simulink model "BESS_GFM_PV_GFL_10kV_Stage1"  (R2026a)
settings: Solver=ode23t  StopTime=0.8  MaxStep=1e-5
InitFcn:
  | run(fullfile(fileparts(get_param(bdroot,'FileName')),'..','scripts','init_bess_pv_stage1.m'));
undefined symbols (not defined in the file): ee_sli_rtmsupport, G, gcbh, S1
libraries: ee_lib x19, nesl_utility x15, fl_lib x14, eeGeneralControl x4, simulink x3, eeTransforms x2, sl_discontinuities x1, sl_signal_attributes x1
(part 1 of 2)
settings Model: Creator=fakebob2004  LastModifiedBy=fakebob2004
settings SimscapeCC: SimscapeLogType=none

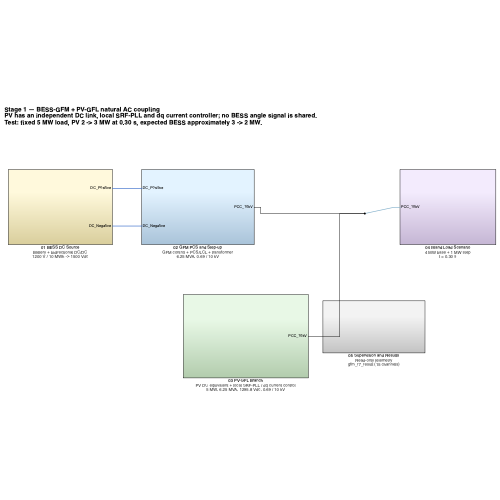
[thumbnail: Simulink's stored preview of the top-level diagram]
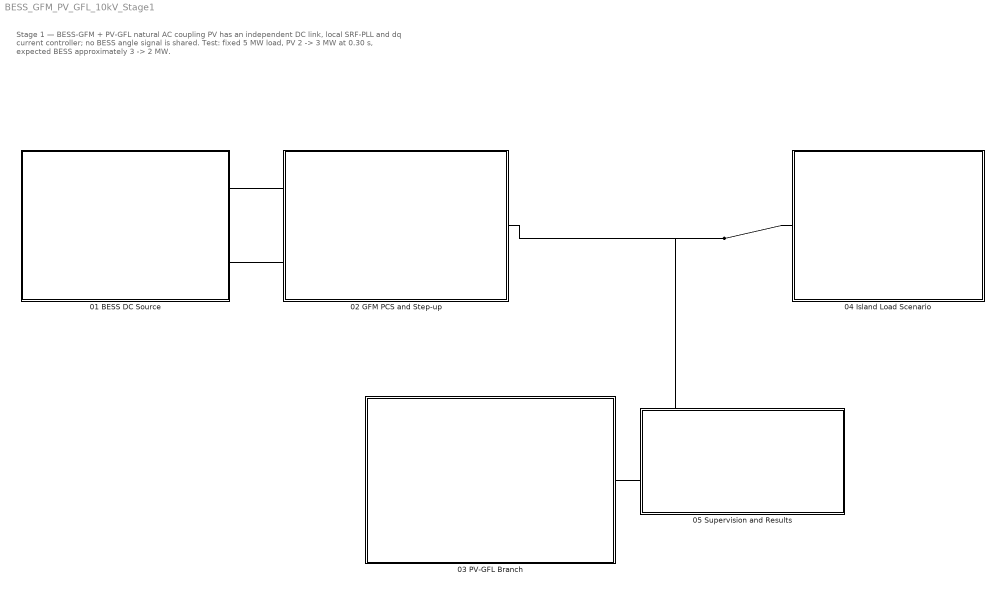
== system BESS_GFM_PV_GFL_10kV_Stage1 ==
  note: Stage 1 — BESS-GFM + PV-GFL natural AC coupling
      | PV has an independent DC link, local SRF-PLL and dq current controller; no BESS angle signal is shared.
      | Test: fixed 5 MW load, PV 2 -> 3 MW at 0.30 s, expected BESS approximately 3 -> 2 MW.
  01 BESS DC Source : Subsystem
      settings: AttributesFormatString=Battery + bidirectional DC/DC\n1200 V / 10 MWh -> 1500 Vdc
  02 GFM PCS and Step-up : Subsystem
      settings: AttributesFormatString=GFM control + PCS/LCL + transformer\n6.25 MVA, 0.69 / 10 kV
  03 PV-GFL Branch : Subsystem
      settings: AttributesFormatString=|
      | PV DC equivalent + local SRF-PLL / dq current control
      | 5 MW, 6.25 MVA, 1295.8 Vdc, 0.69 / 10 kV
  04 Island Load Scenario : Subsystem
      settings: AttributesFormatString=4 MW base + 1 MW step\nt = 0.30 s
  05 Supervision and Results : Subsystem
      settings: AttributesFormatString=Read-only telemetry\ngfm_r7_result (15 channels)
  connections:
  01 BESS DC Source/RConn1 -- 02 GFM PCS and Step-up/LConn1
  01 BESS DC Source/RConn2 -- 02 GFM PCS and Step-up/LConn2
  04 Island Load Scenario/LConn1 -- 02 GFM PCS and Step-up/RConn1 -- 03 PV-GFL Branch/RConn1

== system BESS_GFM_PV_GFL_10kV_Stage1/01 BESS DC Source ==
  01 Battery and DC Link : Subsystem
      settings: AttributesFormatString=1200 V / 10 MWh\n1500 V DC link
  02 Bidirectional DC-DC Control : Subsystem
      settings: AttributesFormatString=Vdc PI: 10 Hz\nIbat PI: 300 Hz
  DC_Positive : PMIOPort  Side=Right  ConnectionType=Connection: foundation.electrical.electrical
  DC_Negative : PMIOPort  Port=2  Side=Right  ConnectionType=Connection: foundation.electrical.electrical
  connections:
  02 Bidirectional DC-DC Control/RConn1 -- 01 Battery and DC Link/LConn2
  01 Battery and DC Link/RConn2 -- DC_Negative/RConn1
  DC_Positive/RConn1 -- 01 Battery and DC Link/LConn1

== system BESS_GFM_PV_GFL_10kV_Stage1/02 GFM PCS and Step-up ==
  03 GFM Control and Limits : Subsystem
      settings: AttributesFormatString=P-f / Q-V / Virtual Z\nAC limit: 1.20 pu
  04 PCS Filter and Transformer : Subsystem
      settings: AttributesFormatString=6.25 MVA PCS + LCL\n0.69 / 10 kV transformer
  DC_Positive : PMIOPort  Side=Left  ConnectionType=Connection: foundation.electrical.electrical
  DC_Negative : PMIOPort  Port=2  Side=Left  ConnectionType=Connection: foundation.electrical.electrical
  PCC_10kV : PMIOPort  Port=3  Side=Right  ConnectionType=Connection: foundation.electrical.three_phase
  connections:
  04 PCS Filter and Transformer/RConn3 -- DC_Negative/RConn1
  04 PCS Filter and Transformer/RConn2 -- PCC_10kV/RConn1
  04 PCS Filter and Transformer/RConn1 -- DC_Positive/RConn1
  03 GFM Control and Limits/RConn1 -- 04 PCS Filter and Transformer/LConn1

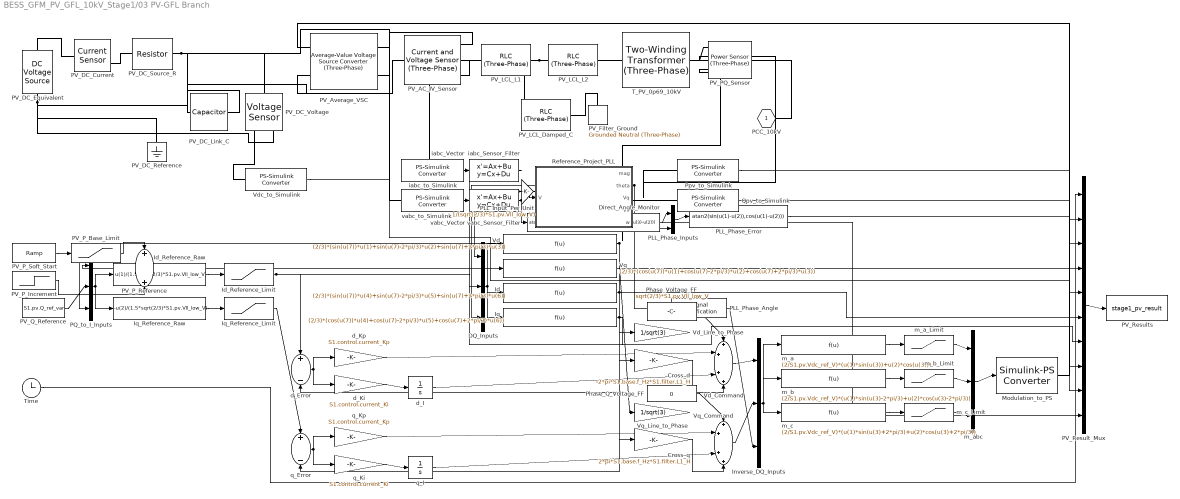
== system BESS_GFM_PV_GFL_10kV_Stage1/03 PV-GFL Branch ==
  Cross_d : Gain  Gain=-2*pi*S1.base.f_Hz*S1.filter.L1_H
  Cross_q : Gain  Gain=2*pi*S1.base.f_Hz*S1.filter.L1_H
  DQ_Inputs : Mux  Inputs=3
  Direct_Angle_Monitor : Fcn  Expr=atan2((2/3)*(u(1)-0.5*u(2)-0.5*u(3)),(sqrt(3)/3)*(u(3)-u(2)))
  Id : Fcn  Expr=(2/3)*(sin(u(7))*u(4)+sin(u(7)-2*pi/3)*u(5)+sin(u(7)+2*pi/3)*u(6))
  Id_Reference_Limit : Saturate  UpperLimit=S1.control.Ilimit_A  LowerLimit=-S1.control.Ilimit_A
  Id_Reference_Raw : Fcn  Expr=u(1)/(1.5*sqrt(2/3)*S1.pv.Vll_low_V)
  Inverse_DQ_Inputs : Mux  Inputs=3
  Iq : Fcn  Expr=(2/3)*(cos(u(7))*u(4)+cos(u(7)-2*pi/3)*u(5)+cos(u(7)+2*pi/3)*u(6))
  Iq_Reference_Limit : Saturate  UpperLimit=S1.control.Ilimit_A  LowerLimit=-S1.control.Ilimit_A
  Iq_Reference_Raw : Fcn  Expr=-u(2)/(1.5*sqrt(2/3)*S1.pv.Vll_low_V)
  Modulation_to_PS : nesl_utility/Simulink-PS Converter  PhysicalDomain=network_engine_domain  SubClassName=ps_input  LeftPortType=input  RightPortType=output  PseudoPeriodic=off  Frequencies=[]  NoiseDistribution=none  NoiseParameters=[]  Unit=1  AffineConversion=off  FilteringAndDerivatives=zero  SimscapeFilterOrder=1  InputFilterTimeConstant=0.001  UdotUserProvided=0
  PLL_Input_Per_Unit : Gain  Gain=1/(sqrt(2/3)*S1.pv.Vll_low_V)
  PLL_Phase_Angle : SignalSpecification
  PLL_Phase_Error : Fcn  Expr=atan2(sin(u(1)-u(2)),cos(u(1)-u(2)))
  PLL_Phase_Inputs : Mux  Inputs=2
  PQ_to_I_Inputs : Mux  Inputs=3
  PV_AC_IV_Sensor : ee_lib/Sensors & Transducers/Current and Voltage Sensor (Three-Phase)  port_option=ee.enum.threePhasePort.composite  vMeasurementType=ee.enum.vmeasurement.ll  outputUnit=ee.enum.unit.si  SRated=100e6 A*V  VRated=24e3 V  I_specify=off  I_priority=None  I=[0, 0, 0] A  I_nominal_specify=off  I_nominal_value=1  I_nominal_unit=A  V_specify=off  V_priority=None  V=[0, 0, 0] V  V_nominal_specify=off  V_nominal_value=1  V_nominal_unit=V
  PV_Average_VSC : ee_lib/Semiconductors & Converters/Converters/Average-Value Voltage Source Converter (Three-Phase)  port_option=ee.enum.threePhasePort.composite  enable_block_pulses_input=false  krec=0.001 Ohm  frequency_option=ee.enum.converters.frequency.variable  input_option=ee.enum.converters.inputOption.ModWave  FRated=S1.base.f_Hz Hz  losses_parameterization=ee.enum.converters.losses.fixed  Pfixed=1 W  ks=0.01  kc1=1.7 V  kc2=0.01 Ohm  Ploss_vect=[100, 800, 1870, 3250, 4900] W  Irms_vect=[10, 100, 200, 300, 400] A  Vdc_nom=300 V  thermal_mass=30000 J/K  temperature_specify=off  temperature_priority=High  temperature=298.15 K  temperature_nominal_specify=off  temperature_nominal_value=1  temperature_nominal_unit=K
  PV_DC_Current : fl_lib/Electrical/Electrical Sensors/Current Sensor
  PV_DC_Equivalent : fl_lib/Electrical/Electrical Sources/DC Voltage Source  v0=S1.pv.Vdc_ref_V V
  PV_DC_Link_C : fl_lib/Electrical/Electrical Elements/Capacitor  c=S1.pv.Cdc_F F  r=1e-6 Ohm  g=0 1/Ohm  i_specify=off  i_priority=None  i=0 A  i_nominal_specify=off  i_nominal_value=1  i_nominal_unit=A  v_specify=off  v_priority=None  v=0 V  v_nominal_specify=off  v_nominal_value=1  v_nominal_unit=V  vc_specify=on  vc_priority=High  vc=S1.pv.Vdc_ref_V V  vc_nominal_specify=off  vc_nominal_value=1  vc_nominal_unit=V
  PV_DC_Reference : fl_lib/Electrical/Electrical Elements/Electrical Reference
  PV_DC_Source_R : fl_lib/Electrical/Electrical Elements/Resistor  R=S1.pv.dc_source_R_ohm Ohm  i_specify=off  i_priority=None  i=0 A  i_nominal_specify=off  i_nominal_value=1  i_nominal_unit=A  v_specify=off  v_priority=None  v=0 V  v_nominal_specify=off  v_nominal_value=1  v_nominal_unit=V
  PV_DC_Voltage : fl_lib/Electrical/Electrical Sensors/Voltage Sensor
  PV_Filter_Ground : ee_lib/Connectors & References/Grounded Neutral (Three-Phase)  port_option=ee.enum.threePhasePort.composite
  PV_LCL_Damped_C : ee_lib/Passive/RLC Assemblies/RLC (Three-Phase)  port_option=ee.enum.threePhasePort.composite  component_structure=ee.enum.rlc.structure.SeriesRC  R=S1.filter.Rd_ohm Ohm  L=1e-3 H  C=S1.filter.C_F F  R_parasitic=0 Ohm  G_parasitic=0 1/Ohm  IL_specify=off  IL_priority=High  IL=[0, 0, 0] A  IL_nominal_specify=off  IL_nominal_value=1  IL_nominal_unit=A  VC_specify=off  VC_priority=High  VC=[0, 0, 0] V  VC_nominal_specify=off  VC_nominal_value=1  VC_nominal_unit=V
  PV_LCL_L1 : ee_lib/Passive/RLC Assemblies/RLC (Three-Phase)  port_option=ee.enum.threePhasePort.composite  component_structure=ee.enum.rlc.structure.SeriesRL  R=S1.filter.R1_ohm Ohm  L=S1.filter.L1_H H  C=1e-6 F  R_parasitic=0 Ohm  G_parasitic=0 1/Ohm  IL_specify=off  IL_priority=High  IL=[0, 0, 0] A  IL_nominal_specify=off  IL_nominal_value=1  IL_nominal_unit=A  VC_specify=off  VC_priority=High  VC=[0, 0, 0] V  VC_nominal_specify=off  VC_nominal_value=1  VC_nominal_unit=V
  PV_LCL_L2 : ee_lib/Passive/RLC Assemblies/RLC (Three-Phase)  port_option=ee.enum.threePhasePort.composite  component_structure=ee.enum.rlc.structure.SeriesRL  R=S1.filter.R2_ohm Ohm  L=S1.filter.L2_H H  C=1e-6 F  R_parasitic=0 Ohm  G_parasitic=0 1/Ohm  IL_specify=off  IL_priority=High  IL=[0, 0, 0] A  IL_nominal_specify=off  IL_nominal_value=1  IL_nominal_unit=A  VC_specify=off  VC_priority=High  VC=[0, 0, 0] V  VC_nominal_specify=off  VC_nominal_value=1  VC_nominal_unit=V
  PV_PQ_Sensor : ee_lib/Sensors & Transducers/Power Sensor (Three-Phase)  port_option=ee.enum.threePhasePort.composite  load_type=ee.enum.passive.type_balanced.balanced  f0=60 Hz
  PV_P_Base_Limit : Saturate  UpperLimit=S1.pv.P_initial_W  LowerLimit=0
  PV_P_Increment : Step  Time=S1.pv.P_step_time_s  FinalValue=S1.pv.P_final_W-S1.pv.P_initial_W  SampleTime=0
  PV_P_Reference : Sum
  PV_P_Soft_Start : simulink/Sources/Ramp  slope=S1.pv.P_ramp_W_per_s  start=0  InitialOutput=0
  PV_Q_Reference : Constant  Value=S1.pv.Q_ref_var
  PV_Result_Mux : Mux  Inputs=10
  PV_Results : ToWorkspace  VariableName=stage1_pv_result  SampleTime=-1
  Phase_Q_Voltage_FF : Constant  Value=0
  Phase_Voltage_FF : Constant  Value=sqrt(2/3)*S1.pv.Vll_low_V
  Ppv_to_Simulink : nesl_utility/PS-Simulink Converter  PhysicalDomain=network_engine_domain  SubClassName=ps_output  LeftPortType=input  RightPortType=output  PseudoPeriodic=off  Frequencies=[]  VectorFormat=inherit  Unit=W  AffineConversion=off
  Qpv_to_Simulink : nesl_utility/PS-Simulink Converter  PhysicalDomain=network_engine_domain  SubClassName=ps_output  LeftPortType=input  RightPortType=output  PseudoPeriodic=off  Frequencies=[]  VectorFormat=inherit  Unit=W  AffineConversion=off
  Reference_Project_PLL : Subsystem
      settings: PortSchema="{\"entries\":[{\"content\":{\"sides\":[{\"content\":{\"connectorIds\":[\"Out1\",\"Out2\",\"Out3\",\"Out4\",\"Out5\"]},\"type\":\"ConnectorPlacement.EquallySpacedRectSide\",\"uuid\":\"76485780-20fe-4fcf-8224-69648da6ed2a\"},{\"content\":{\"connectorIds\":[\"In1\"],\"side\":\"RIGHT\"},\"type\":\"ConnectorPlacement.EquallySpacedRectSide\",\"uuid\":\"f19a6390-e634-42c7-8d46-4cd80cbab182\"},{\"content\":{\"side\":\"TOP\"},\"type\":\"ConnectorPlacement.EquallySpacedRectSide\",\"uuid\":\"87682f72-1844-428e-be70-ad7ca3191ee3\"}]},\"type\":\"ConnectorPlacement.EquallySpacedConnector\",\"uuid\":\"f2136b07-48ec-402b-adb3-18c0bac2157c\"}],\"packageUris\":[\"http://schema.mathworks.com/mf0/Connector/R2020b\"],\"version\":\"1.0\"}"
  T_PV_0p69_10kV : ee_lib/Passive/Transformers/Two-Winding Transformer (Three-Phase)  SRated=S1.transformer.S_VA A*V  FRated=S1.base.f_Hz Hz  Winding1Connection=ee.enum.windingconnection.delta1  VRated1=S1.pv.Vll_low_V V  Winding2Connection=ee.enum.windingconnection.Yg  VRated2=S1.pv.Vll_high_V V  CoreType=ee.enum.coretype.threelimb  pu_Rw1=S1.transformer.R_pu/2  pu_Rw2=S1.transformer.R_pu/2  leakage_reactance_option=ee.enum.transformer_leakage.include  pu_Xl1=S1.transformer.X_pu/2  pu_Xl2=S1.transformer.X_pu/2  magnetizing_resistance_option=ee.enum.transformer_magnetizingResistance.exclude  pu_Rm=500  magnetizing_reactance_option=ee.enum.transformer_magnetizingReactance.exclude  saturation_option=ee.enum.transformer_saturation.exclude  pu_Xm=500  current_data=[0, .002, 1, 2]  magnetic_flux_data=[0, 1.2, 1.5, 1.51]  pu_X0=0.5  i1_specify=off  i1_priority=None  i1=[0, 0, 0] A  i1_nominal_specify=off  i1_nominal_value=1  i1_nominal_unit=A  i2_specify=off  i2_priority=None  i2=[0, 0, 0] A  i2_nominal_specify=off  i2_nominal_value=1  i2_nominal_unit=A  phi_specify=off  phi_priority=None  phi=[0, 0, 0]  phi_nominal_specify=off  phi_nominal_value=1  phi_nominal_unit=1
  Time : Clock
  Vd : Fcn  Expr=(2/3)*(sin(u(7))*u(1)+sin(u(7)-2*pi/3)*u(2)+sin(u(7)+2*pi/3)*u(3))
  Vd_Command : Sum  Inputs=++++
  Vd_Line_to_Phase : Gain  Gain=1/sqrt(3)
  Vdc_to_Simulink : nesl_utility/PS-Simulink Converter  PhysicalDomain=network_engine_domain  SubClassName=ps_output  LeftPortType=input  RightPortType=output  PseudoPeriodic=off  Frequencies=[]  VectorFormat=inherit  Unit=V  AffineConversion=off
  Vq : Fcn  Expr=(2/3)*(cos(u(7))*u(1)+cos(u(7)-2*pi/3)*u(2)+cos(u(7)+2*pi/3)*u(3))
  Vq_Command : Sum  Inputs=++++
  Vq_Line_to_Phase : Gain  Gain=1/sqrt(3)
  d_Error : Sum  Inputs=+-
  d_I : Integrator
  d_Ki : Gain  Gain=S1.control.current_Ki
  d_Kp : Gain  Gain=S1.control.current_Kp
  iabc_Sensor_Filter : StateSpace  A=-eye(3)/S1.control.sensor_filter_s  B=eye(3)/S1.control.sensor_filter_s  C=eye(3)  D=zeros(3)  InitialCondition=zeros(3,1)
  iabc_Vector : Reshape
  iabc_to_Simulink : nesl_utility/PS-Simulink Converter  PhysicalDomain=network_engine_domain  SubClassName=ps_output  LeftPortType=input  RightPortType=output  PseudoPeriodic=off  Frequencies=[]  VectorFormat=inherit  Unit=A  AffineConversion=off
  m_a : Fcn  Expr=(2/S1.pv.Vdc_ref_V)*(u(1)*sin(u(3))+u(2)*cos(u(3)))
  m_a_Limit : Saturate  UpperLimit=S1.pv.modulation_max  LowerLimit=-S1.pv.modulation_max
  m_abc : Mux  Inputs=3
  m_b : Fcn  Expr=(2/S1.pv.Vdc_ref_V)*(u(1)*sin(u(3)-2*pi/3)+u(2)*cos(u(3)-2*pi/3))
  m_b_Limit : Saturate  UpperLimit=S1.pv.modulation_max  LowerLimit=-S1.pv.modulation_max
  m_c : Fcn  Expr=(2/S1.pv.Vdc_ref_V)*(u(1)*sin(u(3)+2*pi/3)+u(2)*cos(u(3)+2*pi/3))
  m_c_Limit : Saturate  UpperLimit=S1.pv.modulation_max  LowerLimit=-S1.pv.modulation_max
  q_Error : Sum  Inputs=+-
  q_I : Integrator
  q_Ki : Gain  Gain=S1.control.current_Ki
  q_Kp : Gain  Gain=S1.control.current_Kp
  vabc_Sensor_Filter : StateSpace  A=-eye(3)/S1.control.sensor_filter_s  B=eye(3)/S1.control.sensor_filter_s  C=eye(3)  D=zeros(3)  InitialCondition=sqrt(2/3)*S1.pv.Vll_low_V*[sin(pi/6);sin(pi/6-2*pi/3);sin(pi/6+2*pi/3)]
  vabc_Vector : Reshape
  vabc_to_Simulink : nesl_utility/PS-Simulink Converter  PhysicalDomain=network_engine_domain  SubClassName=ps_output  LeftPortType=input  RightPortType=output  PseudoPeriodic=off  Frequencies=[]  VectorFormat=inherit  Unit=V  AffineConversion=off
  PCC_10kV : PMIOPort  Side=Right  ConnectionType=Connection: foundation.electrical.three_phase
  wires:
  iabc_to_Simulink/1 -> iabc_Vector/1
  vabc_to_Simulink/1 -> vabc_Vector/1
  iabc_Vector/1 -> iabc_Sensor_Filter/1
  vabc_Vector/1 -> vabc_Sensor_Filter/1
  vabc_Sensor_Filter/1 -> PLL_Input_Per_Unit/1, Direct_Angle_Monitor/1, DQ_Inputs/1
  PLL_Input_Per_Unit/1 -> Reference_Project_PLL/1(V)
  Direct_Angle_Monitor/1 -> PLL_Phase_Inputs/1
  Reference_Project_PLL/2(theta) -> PLL_Phase_Inputs/2, DQ_Inputs/3, PLL_Phase_Angle/1
  PLL_Phase_Inputs/1 -> PLL_Phase_Error/1
  iabc_Sensor_Filter/1 -> DQ_Inputs/2
  DQ_Inputs/1 -> Vd/1, Vq/1, Id/1, Iq/1
  PV_P_Soft_Start/1 -> PV_P_Base_Limit/1
  PV_P_Base_Limit/1 -> PV_P_Reference/1
  PV_P_Increment/1 -> PV_P_Reference/2
  PV_P_Reference/1 -> PQ_to_I_Inputs/1, PV_Result_Mux/4
  PV_Q_Reference/1 -> PQ_to_I_Inputs/2
  Vd/1 -> PQ_to_I_Inputs/3, Vd_Line_to_Phase/1
  PQ_to_I_Inputs/1 -> Id_Reference_Raw/1, Iq_Reference_Raw/1
  Id_Reference_Raw/1 -> Id_Reference_Limit/1
  Iq_Reference_Raw/1 -> Iq_Reference_Limit/1
  d_Error/1 -> d_Kp/1, d_Ki/1
  d_Ki/1 -> d_I/1
  q_Error/1 -> q_Kp/1, q_Ki/1
  q_Ki/1 -> q_I/1
  Id_Reference_Limit/1 -> d_Error/1, PV_Result_Mux/8
  Id/1 -> d_Error/2, Cross_q/1, PV_Result_Mux/6
  Iq_Reference_Limit/1 -> q_Error/1
  Iq/1 -> q_Error/2, Cross_d/1, PV_Result_Mux/7
  Vq/1 -> Vq_Line_to_Phase/1
  Phase_Voltage_FF/1 -> Vd_Command/1
  d_Kp/1 -> Vd_Command/2
  d_I/1 -> Vd_Command/3
  Cross_d/1 -> Vd_Command/4
  Phase_Q_Voltage_FF/1 -> Vq_Command/1
  q_Kp/1 -> Vq_Command/2
  q_I/1 -> Vq_Command/3
  Cross_q/1 -> Vq_Command/4
  Vd_Command/1 -> Inverse_DQ_Inputs/1
  Vq_Command/1 -> Inverse_DQ_Inputs/2
  PLL_Phase_Angle/1 -> Inverse_DQ_Inputs/3
  Inverse_DQ_Inputs/1 -> m_a/1, m_b/1, m_c/1
  m_a/1 -> m_a_Limit/1
  m_b/1 -> m_b_Limit/1
  m_c/1 -> m_c_Limit/1
  m_a_Limit/1 -> m_abc/1
  m_b_Limit/1 -> m_abc/2
  m_c_Limit/1 -> m_abc/3
  m_abc/1 -> Modulation_to_PS/1
  Time/1 -> PV_Result_Mux/1
  Ppv_to_Simulink/1 -> PV_Result_Mux/2
  Qpv_to_Simulink/1 -> PV_Result_Mux/3
  PLL_Phase_Error/1 -> PV_Result_Mux/5
  Vdc_to_Simulink/1 -> PV_Result_Mux/9
  Reference_Project_PLL/5(w) -> PV_Result_Mux/10
  PV_Result_Mux/1 -> PV_Results/1
  connections:
  PV_DC_Equivalent/LConn1 -- PV_DC_Current/LConn1
  PV_DC_Current/RConn2 -- PV_DC_Source_R/LConn1
  PV_Average_VSC/RConn1 -- PV_DC_Source_R/RConn1 -- PV_DC_Link_C/LConn1 -- PV_DC_Voltage/LConn1
  PV_Average_VSC/RConn2 -- PV_DC_Equivalent/RConn1 -- PV_DC_Link_C/RConn1 -- PV_DC_Voltage/RConn2 -- PV_DC_Reference/LConn1
  PV_Average_VSC/LConn2 -- PV_AC_IV_Sensor/LConn1
  PV_AC_IV_Sensor/RConn3 -- PV_LCL_L1/LConn1
  PV_LCL_L2/LConn1 -- PV_LCL_L1/RConn1 -- PV_LCL_Damped_C/LConn1
  PV_LCL_Damped_C/RConn1 -- PV_Filter_Ground/LConn1
  PV_LCL_L2/RConn1 -- T_PV_0p69_10kV/LConn1
  T_PV_0p69_10kV/RConn1 -- PV_PQ_Sensor/LConn1
  PV_PQ_Sensor/RConn1 -- PCC_10kV/RConn1
  PV_AC_IV_Sensor/RConn2 -- iabc_to_Simulink/LConn1
  PV_AC_IV_Sensor/RConn1 -- vabc_to_Simulink/LConn1
  PV_PQ_Sensor/LConn2 -- Ppv_to_Simulink/LConn1
  PV_PQ_Sensor/LConn3 -- Qpv_to_Simulink/LConn1
  PV_DC_Voltage/RConn1 -- Vdc_to_Simulink/LConn1
  Modulation_to_PS/RConn1 -- PV_Average_VSC/LConn1

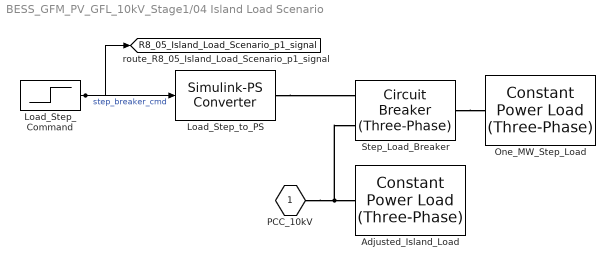
== system BESS_GFM_PV_GFL_10kV_Stage1/04 Island Load Scenario ==
  Adjusted_Island_Load : ee_lib/Passive/Constant Power Load (Three-Phase)  port_option=ee.enum.threePhasePort.composite  FRated=G.f0_Hz Hz  active_power=S1.load.P_W W  reactive_power=S1.load.Q_var V*A  Vline_rms_min=0.70*G.ac.Vll_high_V V  tau=0.01 s  Vline_rms_ini=G.ac.Vll_high_V V  Vang_ini=0 deg  gmin=1e-6 S
  Load_Step_Command : Step  Time=G.load.step_time_s  InitialValue=1  FinalValue=0  SampleTime=0
  Load_Step_to_PS : nesl_utility/Simulink-PS Converter  PhysicalDomain=network_engine_domain  SubClassName=ps_input  LeftPortType=input  RightPortType=output  PseudoPeriodic=off  Frequencies=[]  NoiseDistribution=none  NoiseParameters=[]  Unit=V  AffineConversion=off  FilteringAndDerivatives=zero  SimscapeFilterOrder=1  InputFilterTimeConstant=0.001  UdotUserProvided=0
  One_MW_Step_Load : ee_lib/Passive/Constant Power Load (Three-Phase)  port_option=ee.enum.threePhasePort.composite  FRated=G.f0_Hz Hz  active_power=0 W  reactive_power=0 V*A  Vline_rms_min=0.70*G.ac.Vll_high_V V  tau=0.01 s  Vline_rms_ini=G.ac.Vll_high_V V  Vang_ini=0 deg  gmin=1e-6 S
  Step_Load_Breaker : ee_lib/Switches & Breakers/Circuit Breaker (Three-Phase)  port_option=ee.enum.threePhasePort.composite  control_port_option=ee.enum.controlport.ps  R_closed=0.001 Ohm  G_open=1e-6 1/Ohm  threshold=0.5 V  breaker_behavior=ee.enum.switches.breakerBehavior.zeroCrossingEnable  i_th=1e-8 A
  PCC_10kV : PMIOPort  Side=Left  ConnectionType=Connection: foundation.electrical.three_phase
  tag scope: R8_05_Island_Load_Scenario_p1_signal=global
  wires:
  Load_Step_Command/1 -> Load_Step_to_PS/1, [R8_05_Island_Load_Scenario_p1_signal]  "step_breaker_cmd"
  connections:
  Step_Load_Breaker/RConn1 -- One_MW_Step_Load/LConn1
  PCC_10kV/RConn1 -- Adjusted_Island_Load/LConn1 -- Step_Load_Breaker/LConn2
  Load_Step_to_PS/RConn1 -- Step_Load_Breaker/LConn1

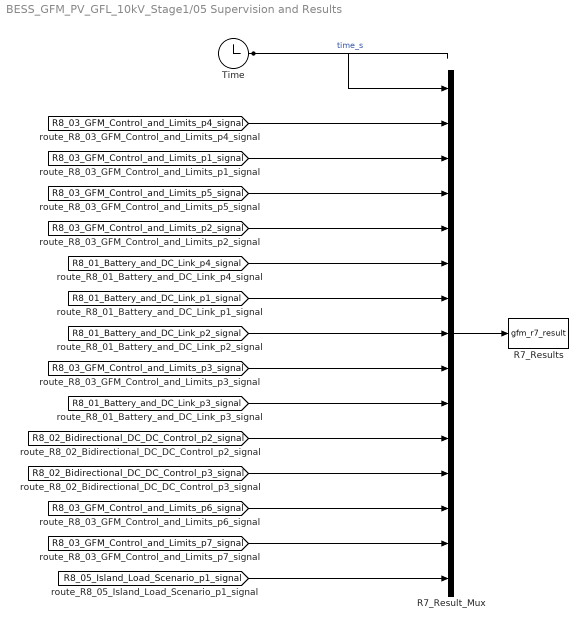
== system BESS_GFM_PV_GFL_10kV_Stage1/05 Supervision and Results ==
  R7_Result_Mux : Mux  Inputs=15
  R7_Results : ToWorkspace  VariableName=gfm_r7_result  SampleTime=-1
  Time : Clock
  wires:
  [R8_05_Island_Load_Scenario_p1_signal] -> R7_Result_Mux/15
  [R8_03_GFM_Control_and_Limits_p7_signal] -> R7_Result_Mux/14
  R7_Result_Mux/1 -> R7_Results/1
  [R8_03_GFM_Control_and_Limits_p6_signal] -> R7_Result_Mux/13
  [R8_02_Bidirectional_DC_DC_Control_p3_signal] -> R7_Result_Mux/12
  [R8_02_Bidirectional_DC_DC_Control_p2_signal] -> R7_Result_Mux/11
  [R8_01_Battery_and_DC_Link_p3_signal] -> R7_Result_Mux/10
  [R8_03_GFM_Control_and_Limits_p3_signal] -> R7_Result_Mux/9
  [R8_01_Battery_and_DC_Link_p2_signal] -> R7_Result_Mux/8
  [R8_01_Battery_and_DC_Link_p1_signal] -> R7_Result_Mux/7
  [R8_01_Battery_and_DC_Link_p4_signal] -> R7_Result_Mux/6
  [R8_03_GFM_Control_and_Limits_p2_signal] -> R7_Result_Mux/5
  Time/1 -> R7_Result_Mux/1  "time_s"
  [R8_03_GFM_Control_and_Limits_p5_signal] -> R7_Result_Mux/4
  [R8_03_GFM_Control_and_Limits_p1_signal] -> R7_Result_Mux/3
  [R8_03_GFM_Control_and_Limits_p4_signal] -> R7_Result_Mux/2

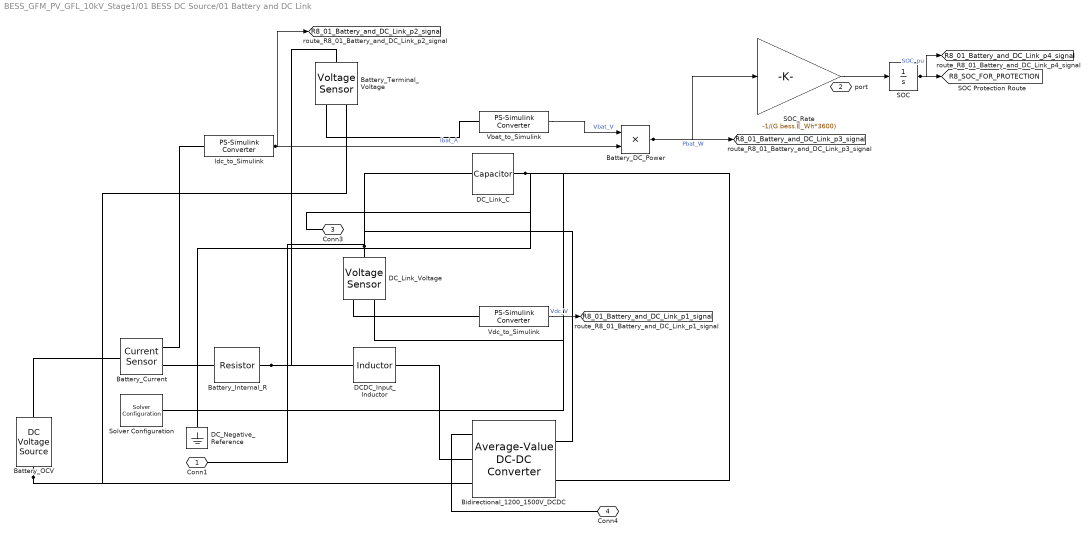
== system BESS_GFM_PV_GFL_10kV_Stage1/01 BESS DC Source/01 Battery and DC Link ==
  Battery_Current : fl_lib/Electrical/Electrical Sensors/Current Sensor
  Battery_DC_Power : Product
  Battery_Internal_R : fl_lib/Electrical/Electrical Elements/Resistor  R=G.dc.Rbattery_ohm Ohm  i_specify=off  i_priority=None  i=0 A  i_nominal_specify=off  i_nominal_value=1  i_nominal_unit=A  v_specify=off  v_priority=None  v=0 V  v_nominal_specify=off  v_nominal_value=1  v_nominal_unit=V
  Battery_OCV : fl_lib/Electrical/Electrical Sources/DC Voltage Source  v0=G.dc.Vbattery_V V
  Battery_Terminal_Voltage : fl_lib/Electrical/Electrical Sensors/Voltage Sensor
  Bidirectional_1200_1500V_DCDC : ee_lib/Semiconductors & Converters/Converters/Average-Value DC-DC Converter  implementation_option=ee.enum.converters.implementation.behavioral  converter_type=ee.enum.converters.dcdctype.buckboost  control_option=ee.enum.converters.controlinput.dutycycle  efficiency_option=ee.enum.converters.efficiency.constant  efficiency_fixed=G.dc.dcdc_efficiency_pct  i_vec=[0, 2, 5] A  efficiency_vec=[90, 95, 98]  Lf=1e-6 H  Rl=0 Ohm  Cf=1e-7 F  Rc=1e-6 Ohm  iL_specify=off  iL_priority=High  iL=0 A  iL_nominal_specify=off  iL_nominal_value=1  iL_nominal_unit=A  vc_specify=off  vc_priority=High  vc=0 V  vc_nominal_specify=off  vc_nominal_value=1  vc_nominal_unit=V
  DCDC_Input_Inductor : fl_lib/Electrical/Electrical Elements/Inductor  l=G.dcdc.L_H H  r=0 Ohm  g=1e-9 1/Ohm  i_specify=on  i_priority=None  i=G.dcdc.Iref_initial_A A  i_nominal_specify=off  i_nominal_value=1  i_nominal_unit=A  v_specify=off  v_priority=None  v=0 V  v_nominal_specify=off  v_nominal_value=1  v_nominal_unit=V  i_L_specify=off  i_L_priority=High  i_L=0 A  i_L_nominal_specify=off  i_L_nominal_value=1  i_L_nominal_unit=A
  DC_Link_C : fl_lib/Electrical/Electrical Elements/Capacitor  c=G.dc.Cdc_F F  r=1e-6 Ohm  g=0 1/Ohm  i_specify=off  i_priority=None  i=0 A  i_nominal_specify=off  i_nominal_value=1  i_nominal_unit=A  v_specify=off  v_priority=None  v=0 V  v_nominal_specify=off  v_nominal_value=1  v_nominal_unit=V  vc_specify=on  vc_priority=High  vc=G.dc.Vdc_ref_V V  vc_nominal_specify=off  vc_nominal_value=1  vc_nominal_unit=V
  DC_Link_Voltage : fl_lib/Electrical/Electrical Sensors/Voltage Sensor
  DC_Negative_Reference : fl_lib/Electrical/Electrical Elements/Electrical Reference
  Idc_to_Simulink : nesl_utility/PS-Simulink Converter  PhysicalDomain=network_engine_domain  SubClassName=ps_output  LeftPortType=input  RightPortType=output  PseudoPeriodic=off  Frequencies=[]  VectorFormat=inherit  Unit=A  AffineConversion=off
  SOC : Integrator  InitialCondition=G.bess.SOC0  LimitOutput=on  UpperSaturationLimit=G.bess.SOC_max  LowerSaturationLimit=G.bess.SOC_min
  SOC_Rate : Gain  Gain=-1/(G.bess.E_Wh*3600)
  Solver Configuration : nesl_utility/Solver Configuration  PhysicalDomain=network_engine_domain  SubClassName=solver  LeftPortType=input  RightPortType=generic  Tones=[]  Harmonics=[]  SimulateNoise=off  Profile=off  UseLocalSampling=off  EnableSwitchedLinearOptims=on  FrequencyDomain=off  UseCCode=off  RelTol=0.001  AbsTol=0.001  MinStep=1e-09  ToWorkspace=off  RevertToSquareIcSolve=off  NumHomotopyIterations=100  PhasorMode=off  PhasorModeNumHarmonics=1  ConsistencySolver=NEWTON_XTOL_AFTER_FTOL  CanonicalOrdering=CANONICAL  OptimizeIntermediates=OPTIMIZED  IndexReductionMethod=DerivativeReplacement  DoDC=off  ResidualTolerance=1e-09  ConsistencyTolSource=GLOBAL  ConsistencyAbsTol=0.001  ConsistencyRelTol=0.001  ConsistencyTolFactor=0.001  UseLocalSolver=off  LocalSolverChoice=NE_BACKWARD_EULER_ADVANCER  ResolveIndetEquations=on  FunctionEvalNumThread=1  LocalSolverSampleTime=0.001  DoFixedCost=off  MaxNonlinIter=3  MaxModeIter=2  ComputeImpulses=off  ImpulseIterations=2  LinearAlgebra=auto  LinearAlgebraNumThread=0  EquationFormulation=NE_TIME_EF  DelaysMemoryBudget=1024  AutomaticFiltering=on  FilteringTimeConstant=0.001  PartitionStorageMethod=AS_NEEDED  PartitionMemoryBudget=1024  PartitionMethod=ROBUST  MultibodyUseLocalSolver=off  MultibodyLocalSolverChoice=ODE1  MultibodyLocalSolverSampleTime=0.001
  Vbat_to_Simulink : nesl_utility/PS-Simulink Converter  PhysicalDomain=network_engine_domain  SubClassName=ps_output  LeftPortType=input  RightPortType=output  PseudoPeriodic=off  Frequencies=[]  VectorFormat=inherit  Unit=V  AffineConversion=off
  Vdc_to_Simulink : nesl_utility/PS-Simulink Converter  PhysicalDomain=network_engine_domain  SubClassName=ps_output  LeftPortType=input  RightPortType=output  PseudoPeriodic=off  Frequencies=[]  VectorFormat=inherit  Unit=V  AffineConversion=off
  Conn1 : PMIOPort  Side=Left
  port : PMIOPort  Port=2  Side=Right
  Conn3 : PMIOPort  Port=3  Side=Right
  Conn4 : PMIOPort  Port=4  Side=Left
  tag scope: R8_01_Battery_and_DC_Link_p1_signal=global, R8_01_Battery_and_DC_Link_p2_signal=global, R8_01_Battery_and_DC_Link_p3_signal=global, R8_01_Battery_and_DC_Link_p4_signal=global, R8_SOC_FOR_PROTECTION=global
  wires:
  SOC/1 -> [R8_01_Battery_and_DC_Link_p4_signal], [R8_SOC_FOR_PROTECTION]  "SOC_pu"
  Battery_DC_Power/1 -> SOC_Rate/1, [R8_01_Battery_and_DC_Link_p3_signal]  "Pbat_W"
  Vbat_to_Simulink/1 -> Battery_DC_Power/1  "Vbat_V"
  Vdc_to_Simulink/1 -> [R8_01_Battery_and_DC_Link_p1_signal]  "Vdc_V"
  SOC_Rate/1 -> SOC/1
  Idc_to_Simulink/1 -> [R8_01_Battery_and_DC_Link_p2_signal], Battery_DC_Power/2  "Ibat_A"
  connections:
  Conn4/RConn1 -- Bidirectional_1200_1500V_DCDC/LConn1
  DC_Link_Voltage/LConn1 -- Bidirectional_1200_1500V_DCDC/RConn1 -- DC_Link_C/LConn1 -- Conn1/RConn1
  Battery_Terminal_Voltage/RConn1 -- Vbat_to_Simulink/LConn1
  DC_Link_Voltage/RConn1 -- Vdc_to_Simulink/LConn1
  Battery_Internal_R/RConn1 -- DCDC_Input_Inductor/LConn1 -- Battery_Terminal_Voltage/LConn1
  Battery_Current/RConn2 -- Battery_Internal_R/LConn1
  DCDC_Input_Inductor/RConn1 -- Bidirectional_1200_1500V_DCDC/LConn2
  Battery_Current/RConn1 -- Idc_to_Simulink/LConn1
  Battery_OCV/LConn1 -- Battery_Current/LConn1
  DC_Negative_Reference/LConn1 -- DC_Link_C/RConn1 -- Bidirectional_1200_1500V_DCDC/RConn2 -- DC_Link_Voltage/RConn2 -- Conn3/RConn1 -- Solver Configuration/RConn1
  Battery_OCV/RConn1 -- Battery_Terminal_Voltage/RConn2 -- Bidirectional_1200_1500V_DCDC/LConn3

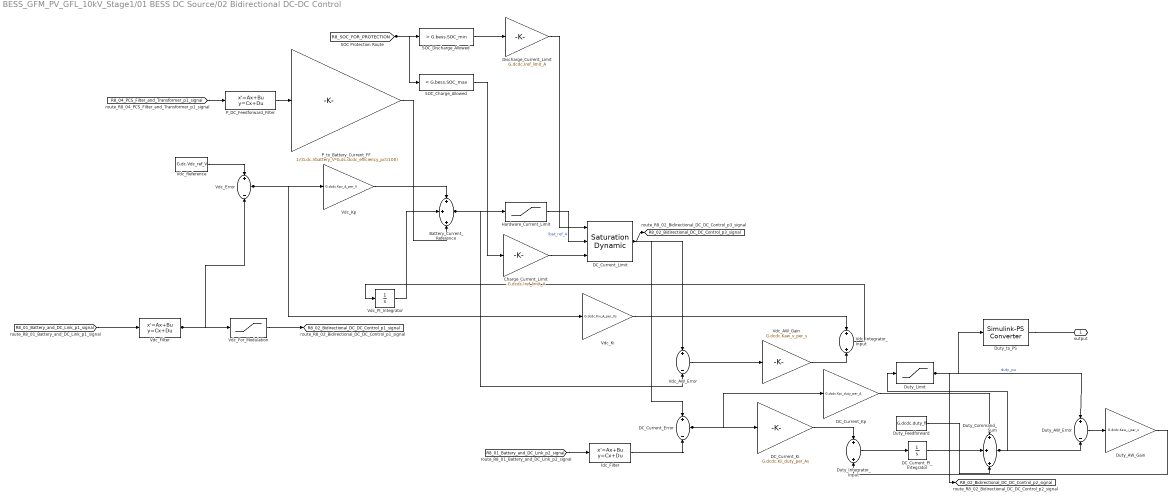
== system BESS_GFM_PV_GFL_10kV_Stage1/01 BESS DC Source/02 Bidirectional DC-DC Control ==
  Battery_Current_Reference : Sum  Inputs=+++
  Charge_Current_Limit : Gain  Gain=-G.dcdc.Iref_limit_A
  DC_Current_Error : Sum  Inputs=+-
  DC_Current_Ki : Gain  Gain=G.dcdc.Kii_duty_per_As
  DC_Current_Kp : Gain  Gain=G.dcdc.Kpi_duty_per_A
  DC_Current_Limit : sl_discontinuities/Saturation Dynamic  OutMin=[]  OutMax=[]  OutDataTypeStr=Inherit: Same as second input  OutDataType=fixdt(1, 16)  OutScaling=2^-10  DoSatur=off
      settings: LibrarySourceBlock=|
      | simulink/Discontinuities/Saturation
      | Dynamic
  DC_Current_PI_Integrator : Integrator
  Discharge_Current_Limit : Gain  Gain=G.dcdc.Iref_limit_A
  Duty_AW_Error : Sum  Inputs=+-
  Duty_AW_Gain : Gain  Gain=G.dcdc.Kaw_i_per_s
  Duty_Command_Sum : Sum  Inputs=+++
  Duty_Feedforward : Constant  Value=G.dcdc.duty_ff
  Duty_Integrator_Input : Sum
  Duty_Limit : Saturate  UpperLimit=G.dcdc.duty_max  LowerLimit=G.dcdc.duty_min
  Duty_to_PS : nesl_utility/Simulink-PS Converter  PhysicalDomain=network_engine_domain  SubClassName=ps_input  LeftPortType=input  RightPortType=output  PseudoPeriodic=off  Frequencies=[]  NoiseDistribution=none  NoiseParameters=[]  Unit=1  AffineConversion=off  FilteringAndDerivatives=zero  SimscapeFilterOrder=1  InputFilterTimeConstant=0.001  UdotUserProvided=0
  Hardware_Current_Limit : Saturate  UpperLimit=G.dcdc.Iref_limit_A  LowerLimit=-G.dcdc.Iref_limit_A
  Idc_Filter : StateSpace  A=-1/G.dcdc.current_sensor_s  B=1/G.dcdc.current_sensor_s  D=0  InitialCondition=G.dcdc.Iref_initial_A
  P_DC_Feedforward_Filter : StateSpace  A=-1/G.dcdc.power_ff_filter_s  B=1/G.dcdc.power_ff_filter_s  D=0  InitialCondition=G.load.base_P_W
  P_to_Battery_Current_FF : Gain  Gain=1/(G.dc.Vbattery_V*G.dc.dcdc_efficiency_pct/100)
  SOC_Charge_Allowed : simulink/Logic and Bit Operations/Compare To Constant  relop=<  const=G.bess.SOC_max  OutDataTypeStr=boolean
  SOC_Discharge_Allowed : simulink/Logic and Bit Operations/Compare To Constant  relop=>  const=G.bess.SOC_min  OutDataTypeStr=boolean
  Vdc_AW_Error : Sum  Inputs=+-
  Vdc_AW_Gain : Gain  Gain=G.dcdc.Kaw_v_per_s
  Vdc_Error : Sum  Inputs=+-
  Vdc_Filter : StateSpace  A=-1/G.control.Vdc_filter_s  B=1/G.control.Vdc_filter_s  D=0  InitialCondition=G.dc.Vdc_ref_V
  Vdc_For_Modulation : Saturate  UpperLimit=2000  LowerLimit=500
  Vdc_Integrator_Input : Sum
  Vdc_Ki : Gain  Gain=G.dcdc.Kiv_A_per_Vs
  Vdc_Kp : Gain  Gain=G.dcdc.Kpv_A_per_V
  Vdc_PI_Integrator : Integrator
  Vdc_Reference : Constant  Value=G.dc.Vdc_ref_V
  output : PMIOPort  Side=Right
  tag scope: R8_02_Bidirectional_DC_DC_Control_p1_signal=global, R8_02_Bidirectional_DC_DC_Control_p2_signal=global, R8_02_Bidirectional_DC_DC_Control_p3_signal=global
  wires:
  Duty_AW_Gain/1 -> Duty_Integrator_Input/2
  Duty_Limit/1 -> [R8_02_Bidirectional_DC_DC_Control_p2_signal], Duty_AW_Error/1, Duty_to_PS/1  "duty_pu"
  Duty_Integrator_Input/1 -> DC_Current_PI_Integrator/1
  DC_Current_Error/1 -> DC_Current_Ki/1, DC_Current_Kp/1
  Idc_Filter/1 -> DC_Current_Error/2
  Discharge_Current_Limit/1 -> DC_Current_Limit/1
  Vdc_Ki/1 -> Vdc_Integrator_Input/1
  SOC_Charge_Allowed/1 -> Charge_Current_Limit/1
  DC_Current_Limit/1 -> [R8_02_Bidirectional_DC_DC_Control_p3_signal], DC_Current_Error/1, Vdc_AW_Error/1
  [R8_01_Battery_and_DC_Link_p2_signal] -> Idc_Filter/1
  Vdc_AW_Error/1 -> Vdc_AW_Gain/1
  Charge_Current_Limit/1 -> DC_Current_Limit/3
  Hardware_Current_Limit/1 -> DC_Current_Limit/2  "Ibat_ref_A"
  Vdc_Integrator_Input/1 -> Vdc_PI_Integrator/1
  Battery_Current_Reference/1 -> Hardware_Current_Limit/1, Vdc_AW_Error/2
  DC_Current_PI_Integrator/1 -> Duty_Command_Sum/2
  SOC_Discharge_Allowed/1 -> Discharge_Current_Limit/1
  Vdc_PI_Integrator/1 -> Battery_Current_Reference/2
  [R8_04_PCS_Filter_and_Transformer_p1_signal] -> P_DC_Feedforward_Filter/1
  Duty_Feedforward/1 -> Duty_Command_Sum/3
  Vdc_For_Modulation/1 -> [R8_02_Bidirectional_DC_DC_Control_p1_signal]
  [R8_SOC_FOR_PROTECTION] -> SOC_Discharge_Allowed/1, SOC_Charge_Allowed/1
  Vdc_Error/1 -> Vdc_Kp/1, Vdc_Ki/1
  Duty_AW_Error/1 -> Duty_AW_Gain/1
  Vdc_AW_Gain/1 -> Vdc_Integrator_Input/2
  Vdc_Reference/1 -> Vdc_Error/1
  [R8_01_Battery_and_DC_Link_p1_signal] -> Vdc_Filter/1
  DC_Current_Ki/1 -> Duty_Integrator_Input/1
  P_DC_Feedforward_Filter/1 -> P_to_Battery_Current_FF/1
  Vdc_Kp/1 -> Battery_Current_Reference/1
  DC_Current_Kp/1 -> Duty_Command_Sum/1
  P_to_Battery_Current_FF/1 -> Battery_Current_Reference/3
  Duty_Command_Sum/1 -> Duty_AW_Error/2, Duty_Limit/1
  Vdc_Filter/1 -> Vdc_For_Modulation/1, Vdc_Error/2
  connections:
  Duty_to_PS/RConn1 -- output/RConn1

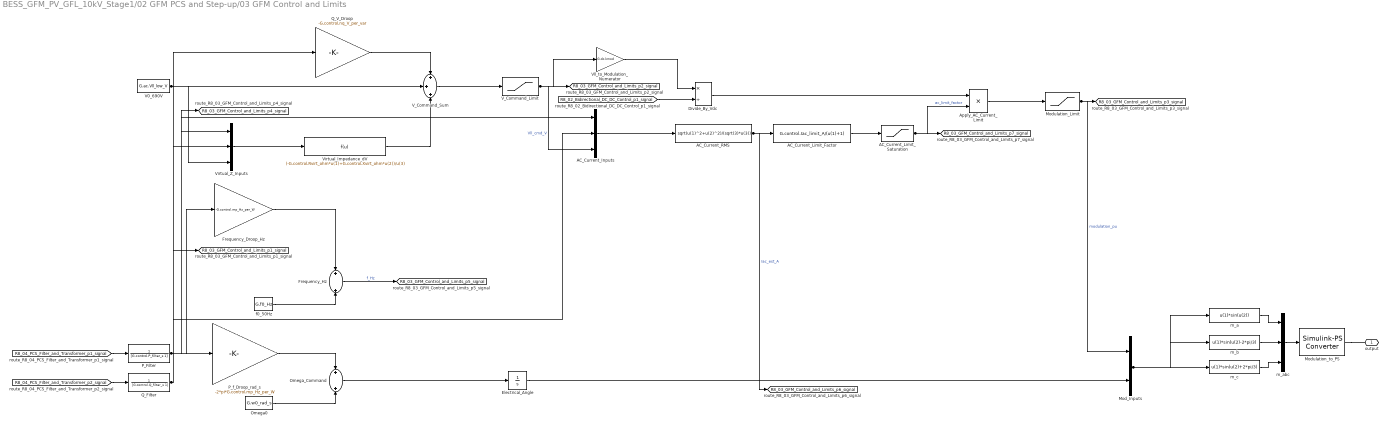
== system BESS_GFM_PV_GFL_10kV_Stage1/02 GFM PCS and Step-up/03 GFM Control and Limits ==
  AC_Current_Inputs : Mux  Inputs=3
  AC_Current_Limit_Factor : Fcn  Expr=G.control.Iac_limit_A/(u(1)+1)
  AC_Current_Limit_Saturation : Saturate  UpperLimit=1  LowerLimit=0
  AC_Current_RMS : Fcn  Expr=sqrt(u(1)^2+u(2)^2)/(sqrt(3)*u(3))
  Apply_AC_Current_Limit : Product
  Divide_By_Vdc : Product  Inputs=*/
  Electrical_Angle : Integrator  InitialCondition=pi/6
  Frequency_Droop_Hz : Gain  Gain=-G.control.mp_Hz_per_W
  Frequency_Hz : Sum
  Mod_Inputs : Mux  Inputs=2
  Modulation_Limit : Saturate  UpperLimit=G.dc.modulation_max  LowerLimit=0
  Modulation_to_PS : nesl_utility/Simulink-PS Converter  PhysicalDomain=network_engine_domain  SubClassName=ps_input  LeftPortType=input  RightPortType=output  PseudoPeriodic=off  Frequencies=[]  NoiseDistribution=none  NoiseParameters=[]  Unit=1  AffineConversion=off  FilteringAndDerivatives=zero  SimscapeFilterOrder=1  InputFilterTimeConstant=0.001  UdotUserProvided=0
  Omega0 : Constant  Value=G.w0_rad_s
  Omega_Command : Sum
  P_Filter : TransferFcn  Numerator=1  Denominator=[G.control.P_filter_s 1]
  P_f_Droop_rad_s : Gain  Gain=-2*pi*G.control.mp_Hz_per_W
  Q_Filter : TransferFcn  Numerator=1  Denominator=[G.control.Q_filter_s 1]
  Q_V_Droop : Gain  Gain=-G.control.nq_V_per_var
  V0_690V : Constant  Value=G.ac.Vll_low_V
  V_Command_Limit : Saturate  UpperLimit=1.10*G.ac.Vll_low_V  LowerLimit=0.90*G.ac.Vll_low_V
  V_Command_Sum : Sum  Inputs=+++
  Virtual_Impedance_dV : Fcn  Expr=(-G.control.Rvirt_ohm*u(1)+G.control.Xvirt_ohm*u(2))/u(3)
  Virtual_Z_Inputs : Mux  Inputs=3
  Vll_to_Modulation_Numerator : Gain  Gain=G.dc.kmod
  f0_50Hz : Constant  Value=G.f0_Hz
  m_a : Fcn  Expr=u(1)*sin(u(2))
  m_abc : Mux  Inputs=3
  m_b : Fcn  Expr=u(1)*sin(u(2)-2*pi/3)
  m_c : Fcn  Expr=u(1)*sin(u(2)+2*pi/3)
  output : PMIOPort  Side=Right
  tag scope: R8_03_GFM_Control_and_Limits_p1_signal=global, R8_03_GFM_Control_and_Limits_p2_signal=global, R8_03_GFM_Control_and_Limits_p3_signal=global, R8_03_GFM_Control_and_Limits_p4_signal=global, R8_03_GFM_Control_and_Limits_p5_signal=global, R8_03_GFM_Control_and_Limits_p6_signal=global, R8_03_GFM_Control_and_Limits_p7_signal=global
  wires:
  m_abc/1 -> Modulation_to_PS/1
  m_c/1 -> m_abc/3
  m_b/1 -> m_abc/2
  Mod_Inputs/1 -> m_a/1, m_b/1, m_c/1
  m_a/1 -> m_abc/1
  Modulation_Limit/1 -> Mod_Inputs/1, [R8_03_GFM_Control_and_Limits_p3_signal]  "modulation_pu"
  AC_Current_Limit_Saturation/1 -> Apply_AC_Current_Limit/2, [R8_03_GFM_Control_and_Limits_p7_signal]  "ac_limit_factor"
  V_Command_Sum/1 -> V_Command_Limit/1
  Divide_By_Vdc/1 -> Apply_AC_Current_Limit/1
  AC_Current_Inputs/1 -> AC_Current_RMS/1
  [R8_02_Bidirectional_DC_DC_Control_p1_signal] -> Divide_By_Vdc/2
  Vll_to_Modulation_Numerator/1 -> Divide_By_Vdc/1
  Apply_AC_Current_Limit/1 -> Modulation_Limit/1
  V_Command_Limit/1 -> Vll_to_Modulation_Numerator/1, AC_Current_Inputs/3, [R8_03_GFM_Control_and_Limits_p2_signal]  "Vll_cmd_V"
  Virtual_Z_Inputs/1 -> Virtual_Impedance_dV/1
  Frequency_Hz/1 -> [R8_03_GFM_Control_and_Limits_p5_signal]  "f_Hz"
  Virtual_Impedance_dV/1 -> V_Command_Sum/3
  Omega0/1 -> Omega_Command/2
  AC_Current_Limit_Factor/1 -> AC_Current_Limit_Saturation/1
  P_f_Droop_rad_s/1 -> Omega_Command/1
  AC_Current_RMS/1 -> AC_Current_Limit_Factor/1, [R8_03_GFM_Control_and_Limits_p6_signal]  "Iac_est_A"
  Q_V_Droop/1 -> V_Command_Sum/1
  f0_50Hz/1 -> Frequency_Hz/2
  P_Filter/1 -> P_f_Droop_rad_s/1, [R8_03_GFM_Control_and_Limits_p4_signal], AC_Current_Inputs/1, Frequency_Droop_Hz/1, Virtual_Z_Inputs/1
  Frequency_Droop_Hz/1 -> Frequency_Hz/1
  Electrical_Angle/1 -> Mod_Inputs/2
  Omega_Command/1 -> Electrical_Angle/1
  [R8_04_PCS_Filter_and_Transformer_p2_signal] -> Q_Filter/1
  V0_690V/1 -> Virtual_Z_Inputs/3, V_Command_Sum/2
  Q_Filter/1 -> [R8_03_GFM_Control_and_Limits_p1_signal], Virtual_Z_Inputs/2, AC_Current_Inputs/2, Q_V_Droop/1
  [R8_04_PCS_Filter_and_Transformer_p1_signal] -> P_Filter/1
  connections:
  Modulation_to_PS/RConn1 -- output/RConn1

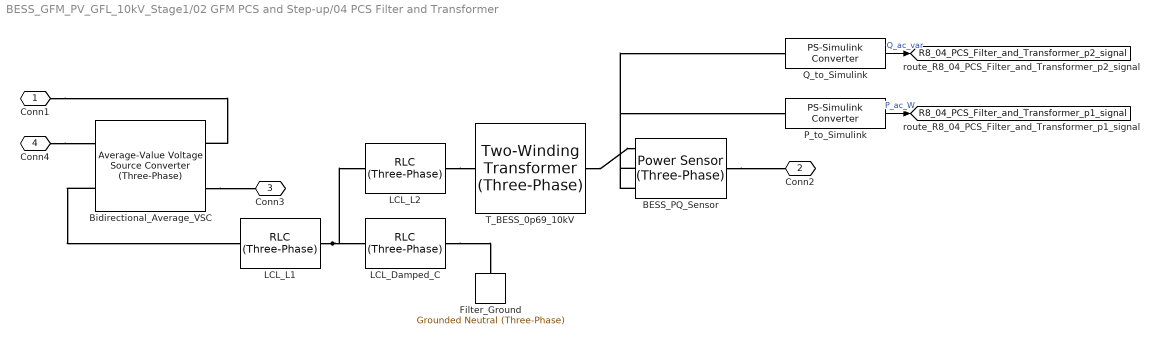
== system BESS_GFM_PV_GFL_10kV_Stage1/02 GFM PCS and Step-up/04 PCS Filter and Transformer ==
  BESS_PQ_Sensor : ee_lib/Sensors & Transducers/Power Sensor (Three-Phase)  port_option=ee.enum.threePhasePort.composite  load_type=ee.enum.passive.type_balanced.balanced  f0=60 Hz
  Bidirectional_Average_VSC : ee_lib/Semiconductors & Converters/Converters/Average-Value Voltage Source Converter (Three-Phase)  port_option=ee.enum.threePhasePort.composite  enable_block_pulses_input=false  krec=G.dc.Rbattery_ohm/10 Ohm  frequency_option=ee.enum.converters.frequency.variable  input_option=ee.enum.converters.inputOption.ModWave  FRated=G.f0_Hz Hz  losses_parameterization=ee.enum.converters.losses.fixed  Pfixed=1 W  ks=0.01  kc1=1.7 V  kc2=0.01 Ohm  Ploss_vect=[100, 800, 1870, 3250, 4900] W  Irms_vect=[10, 100, 200, 300, 400] A  Vdc_nom=300 V  thermal_mass=30000 J/K  temperature_specify=off  temperature_priority=High  temperature=298.15 K  temperature_nominal_specify=off  temperature_nominal_value=1  temperature_nominal_unit=K
  Filter_Ground : ee_lib/Connectors & References/Grounded Neutral (Three-Phase)  port_option=ee.enum.threePhasePort.composite
  LCL_Damped_C : ee_lib/Passive/RLC Assemblies/RLC (Three-Phase)  port_option=ee.enum.threePhasePort.composite  component_structure=ee.enum.rlc.structure.SeriesRC  R=G.filter.Rd_ohm Ohm  L=1e-3 H  C=G.filter.C_F F  R_parasitic=0 Ohm  G_parasitic=0 1/Ohm  IL_specify=off  IL_priority=High  IL=[0, 0, 0] A  IL_nominal_specify=off  IL_nominal_value=1  IL_nominal_unit=A  VC_specify=off  VC_priority=High  VC=[0, 0, 0] V  VC_nominal_specify=off  VC_nominal_value=1  VC_nominal_unit=V
  LCL_L1 : ee_lib/Passive/RLC Assemblies/RLC (Three-Phase)  port_option=ee.enum.threePhasePort.composite  component_structure=ee.enum.rlc.structure.SeriesRL  R=G.filter.R1_ohm Ohm  L=G.filter.L1_H H  C=1e-6 F  R_parasitic=0 Ohm  G_parasitic=0 1/Ohm  IL_specify=off  IL_priority=High  IL=[0, 0, 0] A  IL_nominal_specify=off  IL_nominal_value=1  IL_nominal_unit=A  VC_specify=off  VC_priority=High  VC=[0, 0, 0] V  VC_nominal_specify=off  VC_nominal_value=1  VC_nominal_unit=V
  LCL_L2 : ee_lib/Passive/RLC Assemblies/RLC (Three-Phase)  port_option=ee.enum.threePhasePort.composite  component_structure=ee.enum.rlc.structure.SeriesRL  R=G.filter.R2_ohm Ohm  L=G.filter.L2_H H  C=1e-6 F  R_parasitic=0 Ohm  G_parasitic=0 1/Ohm  IL_specify=off  IL_priority=High  IL=[0, 0, 0] A  IL_nominal_specify=off  IL_nominal_value=1  IL_nominal_unit=A  VC_specify=off  VC_priority=High  VC=[0, 0, 0] V  VC_nominal_specify=off  VC_nominal_value=1  VC_nominal_unit=V
  P_to_Simulink : nesl_utility/PS-Simulink Converter  PhysicalDomain=network_engine_domain  SubClassName=ps_output  LeftPortType=input  RightPortType=output  PseudoPeriodic=off  Frequencies=[]  VectorFormat=inherit  Unit=W  AffineConversion=off
  Q_to_Simulink : nesl_utility/PS-Simulink Converter  PhysicalDomain=network_engine_domain  SubClassName=ps_output  LeftPortType=input  RightPortType=output  PseudoPeriodic=off  Frequencies=[]  VectorFormat=inherit  Unit=W  AffineConversion=off
  T_BESS_0p69_10kV : ee_lib/Passive/Transformers/Two-Winding Transformer (Three-Phase)  SRated=G.transformer.S_VA A*V  FRated=G.f0_Hz Hz  Winding1Connection=ee.enum.windingconnection.delta1  VRated1=G.ac.Vll_low_V V  Winding2Connection=ee.enum.windingconnection.Yg  VRated2=G.ac.Vll_high_V V  CoreType=ee.enum.coretype.threelimb  pu_Rw1=G.transformer.pu_Rw1  pu_Rw2=G.transformer.pu_Rw2  leakage_reactance_option=ee.enum.transformer_leakage.include  pu_Xl1=G.transformer.pu_Xl1  pu_Xl2=G.transformer.pu_Xl2  magnetizing_resistance_option=ee.enum.transformer_magnetizingResistance.exclude  pu_Rm=500  magnetizing_reactance_option=ee.enum.transformer_magnetizingReactance.exclude  saturation_option=ee.enum.transformer_saturation.exclude  pu_Xm=500  current_data=[0, .002, 1, 2]  magnetic_flux_data=[0, 1.2, 1.5, 1.51]  pu_X0=0.5  i1_specify=off  i1_priority=None  i1=[0, 0, 0] A  i1_nominal_specify=off  i1_nominal_value=1  i1_nominal_unit=A  i2_specify=off  i2_priority=None  i2=[0, 0, 0] A  i2_nominal_specify=off  i2_nominal_value=1  i2_nominal_unit=A  phi_specify=off  phi_priority=None  phi=[0, 0, 0]  phi_nominal_specify=off  phi_nominal_value=1  phi_nominal_unit=1
  Conn1 : PMIOPort  Side=Right  ConnectionType=Connection: foundation.electrical.electrical
  Conn2 : PMIOPort  Port=2  Side=Right  ConnectionType=Connection: foundation.electrical.three_phase
  Conn3 : PMIOPort  Port=3  Side=Right  ConnectionType=Connection: foundation.electrical.electrical
  Conn4 : PMIOPort  Port=4  Side=Left
  tag scope: R8_04_PCS_Filter_and_Transformer_p1_signal=global, R8_04_PCS_Filter_and_Transformer_p2_signal=global
  wires:
  P_to_Simulink/1 -> [R8_04_PCS_Filter_and_Transformer_p1_signal]  "P_ac_W"
  Q_to_Simulink/1 -> [R8_04_PCS_Filter_and_Transformer_p2_signal]  "Q_ac_var"
  connections:
  BESS_PQ_Sensor/RConn1 -- Conn2/RConn1
  BESS_PQ_Sensor/LConn3 -- Q_to_Simulink/LConn1
  LCL_Damped_C/RConn1 -- Filter_Ground/LConn1
  LCL_L2/RConn1 -- T_BESS_0p69_10kV/LConn1
  Bidirectional_Average_VSC/RConn2 -- Conn3/RConn1
  LCL_L1/RConn1 -- LCL_L2/LConn1 -- LCL_Damped_C/LConn1
  T_BESS_0p69_10kV/RConn1 -- BESS_PQ_Sensor/LConn1
  Bidirectional_Average_VSC/LConn2 -- LCL_L1/LConn1
  Conn4/RConn1 -- Bidirectional_Average_VSC/LConn1
  BESS_PQ_Sensor/LConn2 -- P_to_Simulink/LConn1
  Conn1/RConn1 -- Bidirectional_Average_VSC/RConn1

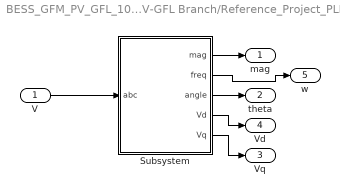
== system BESS_GFM_PV_GFL_10kV_Stage1/03 PV-GFL Branch/Reference_Project_PLL ==
  V : Inport
  Subsystem : Subsystem
  mag : Outport
  theta : Outport  Port=2
  Vq : Outport  Port=3
  Vd : Outport  Port=4
  w : Outport  Port=5
  wires:
  Subsystem/2(freq) -> w/1
  Subsystem/4(Vd) -> Vd/1
  Subsystem/5(Vq) -> Vq/1
  Subsystem/3(angle) -> theta/1
  Subsystem/1(mag) -> mag/1
  V/1 -> Subsystem/1(abc)

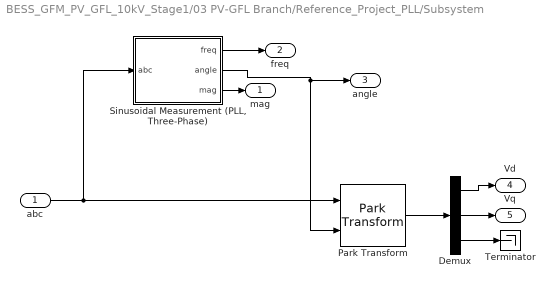
== system BESS_GFM_PV_GFL_10kV_Stage1/03 PV-GFL Branch/Reference_Project_PLL/Subsystem ==
  abc : Inport
  Demux : Demux  Outputs=3
  Park Transform : eeTransforms/Park Transform  AxisAlignment=Q-axis  PowerInvariant=off
  "Sinusoidal Measurement (PLL, Three-Phase)" : Subsystem  LoadFcn=ee_sli_rtmsupport( 'loadfcn', gcbh );  mask(Sinusoidal Measurement (PLL, Three-Phase)){InputFilter=on, InputNormalization=off, Kp_LF=S1.control.pll_Kp, Ki_LF=S1.control.pll_Ki, F0=S1.base.f_Hz, Theta0=S1.control.pll_initial_phase_rad, Ts=S1.control.pll_sample_s}
      mask prompts: InputFilter "physmod:ee:library:comments:control:eeSinusoidalMeasurement:EnableMovingAverageFilterOnInput_MP"; InputNormalization "physmod:ee:library:comments:control:eeSinusoidalMeasurement:EnableInputNormalization_MP"; Kp_LF "physmod:ee:library:comments:control:eeSinusoidalMeasurement:LoopFilterProportionalGain_MP"; Ki_LF "physmod:ee:library:comments:control:eeSinusoidalMeasurement:LoopFilterIntegralGain_MP"; F0 "physmod:ee:library:comments:control:eeSinusoidalMeasurement:InitialFrequencyHz_MP"; Theta0 "physmod:ee:library:comments:control:eeSinusoidalMeasurement:InitialPhaseAnglerad_MP"; Ts "physmod:ee:library:comments:control:eeSinusoidalMeasurement:SampleTime1ForInherited_MP"
      mask help: physmod:ee:library:comments:control:eeSinusoidalMeasurement:SinusoidalPowerMeasurementPLLThreePhase_MD
      mask init:
      | timeDomain = ee.mask.initializeThreePhaseSinusoidalMeasurementPLL(Ts);
      settings: CopyFcn=ee_sli_rtmsupport( 'copyfcn', gcbh );  DeleteFcn=ee_sli_rtmsupport( 'deletefcn', gcbh );  ModelCloseFcn=ee_sli_rtmsupport( 'modelclosefcn', gcbh );  PostSaveFcn=ee_sli_rtmsupport( 'postsavefcn', gcbh );  PreCopyFcn=ee_sli_rtmsupport( 'precopyfcn', gcbh );  OpenFcn=ee_sli_rtmsupport( 'openfcn', gcbh );  CloseFcn=ee_sli_rtmsupport( 'closefcn', gcbh );  PreDeleteFcn=ee_sli_rtmsupport( 'predeletefcn', gcbh );
      mask Help: web(nesl_help(gcbh))
      mask TypeOptions InputFilter: Input filter/InputFilter
      mask TypeOptions InputNormalization: Normalization/InputNormalization
      mask TypeOptions Ts:
      | Angle/Integrator with
      | Wrapped State
      | (Discrete or Continuous)/Ts | PI/Integrator
      | (Discrete or Continuous)/Ts | Moving Average
      | (Variable Frequency)/Ts | Low-Pass Filter
      | (Discrete or Continuous)/Ts
      mask DialogControl InputFilter Prompt: Enable moving average filter on input
      mask DialogControl InputNormalization Prompt: Enable input normalization
      mask DialogControl Kp_LF Prompt: Loop filter proportional gain
      mask DialogControl Ki_LF Prompt: Loop filter integral gain
      mask DialogControl F0 Prompt: Initial frequency (Hz)
      mask DialogControl Theta0 Prompt: Initial phase angle (rad)
      mask DialogControl Ts Prompt: Sample time (-1 for inherited)
      mask Display: ee.mask.drawThreePhaseSinusoidalMeasurementPLL;
  Terminator : Terminator
  mag : Outport
  freq : Outport  Port=2
  angle : Outport  Port=3
  Vd : Outport  Port=4
  Vq : Outport  Port=5
  wires:
  "Sinusoidal Measurement (PLL, Three-Phase)"/2(angle) -> angle/1, Park Transform/2
  "Sinusoidal Measurement (PLL, Three-Phase)"/3(mag) -> mag/1
  "Sinusoidal Measurement (PLL, Three-Phase)"/1(freq) -> freq/1
  Demux/2 -> Vq/1
  Demux/1 -> Vd/1
  Park Transform/1 -> Demux/1
  abc/1 -> "Sinusoidal Measurement (PLL, Three-Phase)"/1(abc), Park Transform/1
  Demux/3 -> Terminator/1

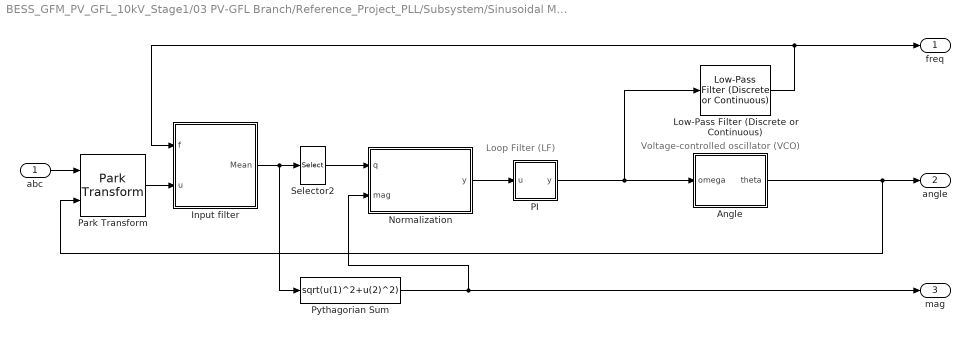
== system BESS_GFM_PV_GFL_10kV_Stage1/03 PV-GFL Branch/Reference_Project_PLL/Subsystem/Sinusoidal Measurement (PLL, Three-Phase) ==
  note: Loop Filter (LF)
  note: Voltage-controlled oscillator (VCO)
  abc : Inport  PortDimensions=3  SampleTime=Ts
  Angle : Subsystem
  Input filter : Subsystem  Variant=on  VariantControlMode=label  LabelModeActiveChoice=Filter  mask{InputFilter=on}
      mask prompts: InputFilter "physmod:ee:library:comments:control:eeSinusoidalMeasurement:EnableMovingAverageFilterOnInput_MP"
      mask Callback InputFilter:
      | if  strcmp(get_param(gcb,'InputFilter'),'on')
      |         try
      |             set_param(gcb,'OverrideUsingVariant','Filter');
      |         catch
      |         end
      |     else
      |         try
      |             set_param(gcb,'OverrideUsingVariant','Passthrough');
      |         catch
      |         end
      |     end
      mask DialogControl InputFilter Prompt: Enable moving average filter on input
  Low-Pass Filter (Discrete or Continuous) : eeGeneralControl/Low-Pass Filter (Discrete or Continuous)  K=1/2/pi  T=1e-3  B=inf  A=-inf  init_option=Specify as parameter  x0=F0  Ts=Ts
  Normalization : Subsystem  Variant=on  VariantControlMode=label  LabelModeActiveChoice=Passthrough  mask{InputNormalization=off}
      mask prompts: InputNormalization "physmod:ee:library:comments:control:eeSinusoidalMeasurement:EnableInputNormalization_MP"
      mask Callback InputNormalization:
      | if  strcmp(get_param(gcb,'InputNormalization'),'on')
      |         try
      |             set_param(gcb,'OverrideUsingVariant','Normalize');
      |         catch
      |         end
      |     else
      |         try
      |             set_param(gcb,'OverrideUsingVariant','Passthrough');
      |         catch
      |         end
      |     end
      mask DialogControl InputNormalization Prompt: Enable input normalization
  PI : Subsystem
  Park Transform : eeTransforms/Park Transform  AxisAlignment=Q-axis  PowerInvariant=off
  Pythagorian Sum : Fcn  Expr=sqrt(u(1)^2+u(2)^2)
  Selector2 : Selector  InputPortWidth=3  IndexOptions=Index vector (dialog)  Indices=[2]  OutputSizes=1
  freq : Outport  VectorParamsAs1DForOutWhenUnconnected=off
  angle : Outport  Port=2  VectorParamsAs1DForOutWhenUnconnected=off
  mag : Outport  Port=3  VectorParamsAs1DForOutWhenUnconnected=off
  wires:
  Selector2/1 -> Normalization/1(q)
  Normalization/1(y) -> PI/1(u)
  Input filter/1(Mean) -> Selector2/1, Pythagorian Sum/1
  Low-Pass Filter (Discrete or Continuous)/1 -> freq/1, Input filter/1(f)
  Angle/1(theta) -> angle/1, Park Transform/2
  PI/1(y) -> Angle/1(omega), Low-Pass Filter (Discrete or Continuous)/1
  Park Transform/1 -> Input filter/2(u)
  Pythagorian Sum/1 -> mag/1, Normalization/2(mag)
  abc/1 -> Park Transform/1

== system BESS_GFM_PV_GFL_10kV_Stage1/03 PV-GFL Branch/Reference_Project_PLL/Subsystem/Sinusoidal Measurement (PLL, Three-Phase)/Angle ==
  omega : Inport
  Integrator with Wrapped State (Discrete or Continuous) : eeGeneralControl/Integrator with Wrapped State (Discrete or Continuous)  LabelModeActiveChoice=Discrete  WrappedStateUpperValue=2*pi  WrappedStateLowerValue=0  x0=Theta0  Ts=Ts
  theta : Outport  VectorParamsAs1DForOutWhenUnconnected=off
  wires:
  Integrator with Wrapped State (Discrete or Continuous)/1 -> theta/1
  omega/1 -> Integrator with Wrapped State (Discrete or Continuous)/1

== system BESS_GFM_PV_GFL_10kV_Stage1/03 PV-GFL Branch/Reference_Project_PLL/Subsystem/Sinusoidal Measurement (PLL, Three-Phase)/Input filter ==
  f : Inport
  u : Inport  Port=2
  Filter : Subsystem  VariantControl=Filter
  Passthrough : Subsystem  VariantControl=Passthrough
  Mean : Outport

== system BESS_GFM_PV_GFL_10kV_Stage1/03 PV-GFL Branch/Reference_Project_PLL/Subsystem/Sinusoidal Measurement (PLL, Three-Phase)/Normalization ==
  q : Inport
  mag : Inport  Port=2
  Normalize : Subsystem  VariantControl=Normalize
  Passthrough : Subsystem  VariantControl=Passthrough
  y : Outport

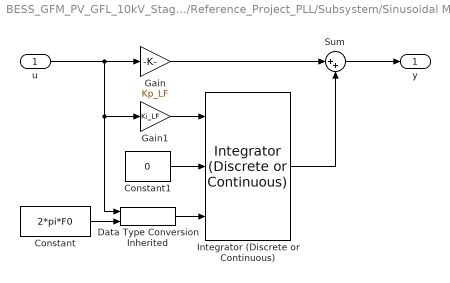
== system BESS_GFM_PV_GFL_10kV_Stage1/03 PV-GFL Branch/Reference_Project_PLL/Subsystem/Sinusoidal Measurement (PLL, Three-Phase)/PI ==
  u : Inport
  Constant : Constant  Value=2*pi*F0  SampleTime=Ts
  Constant1 : Constant  Value=0  SampleTime=Ts
  Data Type Conversion Inherited : sl_signal_attributes/Data Type Conversion Inherited  ConvertRealWorld=Real World Value  DoSatur=off
  Gain : Gain  Gain=Kp_LF
  Gain1 : Gain  Gain=Ki_LF
  Integrator (Discrete or Continuous) : eeGeneralControl/Integrator (Discrete or Continuous)  LabelModeActiveChoice=Discrete  IntegratorMethod=Integration: Forward Euler  ExternalReset=level  LimitType=Anti-windup  B=inf  A=-inf  Ts=Ts
  Sum : Sum  Inputs=|++
  y : Outport  VectorParamsAs1DForOutWhenUnconnected=off
  wires:
  Constant/1 -> Data Type Conversion Inherited/2
  Data Type Conversion Inherited/1 -> Integrator (Discrete or Continuous)/3
  Gain1/1 -> Integrator (Discrete or Continuous)/1
  u/1 -> Gain1/1, Data Type Conversion Inherited/1, Gain/1
  Gain/1 -> Sum/1
  Integrator (Discrete or Continuous)/1 -> Sum/2
  Sum/1 -> y/1
  Constant1/1 -> Integrator (Discrete or Continuous)/2
